simulink model "integrated_controller_scenario5"  (R2021a)
settings: Solver=VariableStepAuto  StartTime=0.0  StopTime=55  RelTol=1e-3
values from neighbouring files (symbols this model uses):
  Cf = 155494.663    [integrated_controller_init.m]    (also in integrated_controller_init_q3.m; integrated_controller_init_q4.m; integrated_controller_init_q5.m; integrated_controller_init_q6_MRM.m)
  Cr = 1554494.663    [integrated_controller_init.m]    (also in integrated_controller_init_q3.m; integrated_controller_init_q4.m; integrated_controller_init_q5.m; integrated_controller_init_q6_MRM.m)
  Iz = 1436.24    [integrated_controller_init.m]    (also in integrated_controller_init_q3.m; integrated_controller_init_q4.m; integrated_controller_init_q5.m; integrated_controller_init_q6_MRM.m)
  L = 3.5    [alc_pathplanning.m]    (also in integrated_controller_init.m = 4.7; integrated_controller_init_q3.m = 4.7; integrated_controller_init_q4.m = 4.7; integrated_controller_init_q5.m = 4.7)
  ld = 10    [integrated_controller_init.m]    (also in integrated_controller_init_q3.m; integrated_controller_init_q4.m; integrated_controller_init_q5.m; integrated_controller_init_q6_MRM.m)
  lf = 1.165    [integrated_controller_init.m]    (also in integrated_controller_init_q3.m; integrated_controller_init_q4.m; integrated_controller_init_q5.m; integrated_controller_init_q6_MRM.m)
  lr = 1.165    [integrated_controller_init.m]    (also in integrated_controller_init_q3.m; integrated_controller_init_q4.m; integrated_controller_init_q5.m; integrated_controller_init_q6_MRM.m)
  m = 1140    [integrated_controller_init.m]    (also in integrated_controller_init_q3.m; integrated_controller_init_q4.m; integrated_controller_init_q5.m; integrated_controller_init_q6_MRM.m)
  md = get_curvature(Vx,yaw_rate_pose,tRef')    [integrated_controller_init.m]    (also in integrated_controller_init_q3.m; integrated_controller_init_q4.m; integrated_controller_init_q5.m; integrated_controller_init_q6_MRM.m)
  Ts = 0.1    [integrated_controller_init.m]    (also in integrated_controller_init_q3.m; integrated_controller_init_q4.m; integrated_controller_init_q5.m; integrated_controller_init_q6_MRM.m)
  V_initial = 15    [integrated_controller_init.m]    (also in integrated_controller_init_q3.m = 11; integrated_controller_init_q4.m = 25; integrated_controller_init_q5.m; integrated_controller_init_q6_MRM.m)
  Vx = a(2) + 2*a(3)*t + 3*a(4)*t.^2 +4*a(5)*t.^3+ a(6)*t.^4    [alc_pathplanning.m]    (also in integrated_controller_init.m = 18; integrated_controller_init_q3.m = 20; integrated_controller_init_q4.m = 25; integrated_controller_init_q5.m = 15)
  xRef = X_ref    [alc_pathplanning.m]    (also in integrated_controller_init.m = path.xRef; integrated_controller_init_q3.m = path.xRef; integrated_controller_init_q4.m = path.xRef; integrated_controller_init_q5.m = refPose(1,:))
  yRef = Y_ref    [alc_pathplanning.m]    (also in integrated_controller_init.m = path.yRef; integrated_controller_init_q3.m = path.yRef; integrated_controller_init_q4.m = path.yRef; integrated_controller_init_q5.m = refPose(2,:))
undefined symbols (not defined in the file or in its folder): sigbuilder_block
libraries: pid_lib x2, mpclib x1, mpcadaslib x1, robotalgslib x1, autolibshared x1
(part 2 of 2)

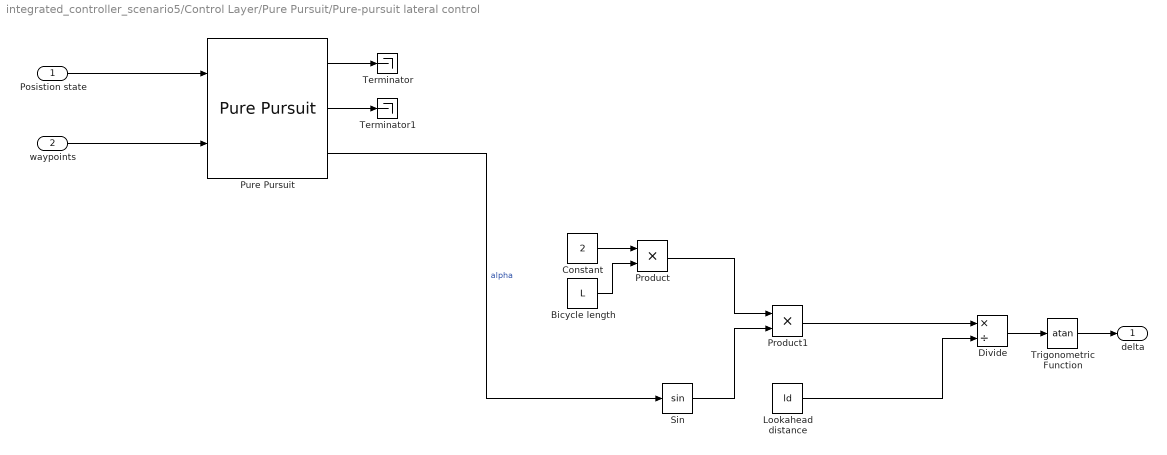
== system integrated_controller_scenario5/Control Layer/Pure Pursuit/Pure-pursuit lateral control ==
  Posistion state : Inport
  waypoints : Inport  Port=2
  Bicycle length : Constant  Value=L
  Constant : Constant  Value=2
  Divide : Product  Inputs=*/
  Lookahead distance : Constant  Value=ld
  Product : Product
  Product1 : Product
  Pure Pursuit : robotalgslib/Pure Pursuit  DesiredLinearVelocity=Vx  MaxAngularVelocity=1.0  LookaheadDistance=ld  TargetDirPort=on  SimulateUsing=Code generation
  Sin : Trigonometry
  Terminator : Terminator
  Terminator1 : Terminator
  Trigonometric Function : Trigonometry  Operator=atan
  delta : Outport
  wires:
  Posistion state/1 -> Pure Pursuit/1
  waypoints/1 -> Pure Pursuit/2
  Pure Pursuit/1 -> Terminator/1
  Pure Pursuit/2 -> Terminator1/1
  Trigonometric Function/1 -> delta/1
  Constant/1 -> Product/1
  Divide/1 -> Trigonometric Function/1
  Lookahead distance/1 -> Divide/2
  Sin/1 -> Product1/2
  Product1/1 -> Divide/1
  Pure Pursuit/3 -> Sin/1  "alpha"
  Bicycle length/1 -> Product/2
  Product/1 -> Product1/1

== system integrated_controller_scenario5/ACC_control_block/ACC_state_logic/Subsystem/If Action Subsystem ==
  v_curve : Inport
  Action Port : ActionPort  ActionPortLabel=if(u1<u2)
  Out1 : Outport
  wires:
  v_curve/1 -> Out1/1

== system integrated_controller_scenario5/ACC_control_block/ACC_state_logic/Subsystem/If Action Subsystem1 ==
  v_limit : Inport
  Action Port : ActionPort  ActionPortLabel=else
  Out1 : Outport
  wires:
  v_limit/1 -> Out1/1

== stateflow chart integrated_controller_scenario5/ACC_control_block/ACC_state_logic/ACC_state_control ==
  state Velocity_and_PSA
    state Velocity_control
      entry: en_man = false;
      en_vel =true;
      en_pos=false;
      en_psa = false;
    state PSA
      entry: en_man = false;
      en_vel =false;
      en_pos=false;
      en_psa = true;
    Velocity_control -> PSA : [v_ideal<v_set]
    (default) -> Velocity_control
    PSA -> Velocity_control : [v_ideal>v_set]
  state Manual_mode
    entry: en_man = true;
    en_vel =false;
    en_pos=false;
  state Headway_control
    entry: en_man = false;
    en_vel =false;
    en_pos=true;
  Manual_mode -> Velocity_and_PSA [order 1] : [(ACC_enable ==1)&&(target_flag==0)]
  Velocity_and_PSA -> Headway_control [order 2] : [(ACC_enable == 1)&(target_flag == 1)&&after(30,sec)]
  Manual_mode -> Headway_control [order 2] : [(ACC_enable == 1) && (target_flag == 1)]
  (default) -> Manual_mode
  Velocity_and_PSA -> Manual_mode [order 1] : [ACC_enable == 0]
  Headway_control -> Velocity_and_PSA [order 2] : [((ACC_enable == 1)&(target_flag==0)|| V_host>commanded_speed + 0.5)&&after(20,sec)]
  Headway_control -> Manual_mode [order 1] : [ACC_enable ==0]
  data: ACC_enable input; V_host input; commanded_speed input; target_flag input; en_man output; en_pos output; en_vel output; en_psa output; v_set input; v_ideal input

== matlab function integrated_controller_scenario5/ACC_control_block/Predictive Speed Assist /MATLAB Function ==
  data: v_limit input; a_max output; v_current input
function a_max = fcn(v_limit,v_current)

if v_current < v_limit+0.2
    a_max = 2000; %mpss
elseif v_current>v_limit+0.2
    a_max = -2000 ; %mpss
else 
    a_max = 0;
    
end

== matlab function integrated_controller_scenario5/Control Layer/MPC/Subsystem/MATLAB Function ==
  settings: updateMethod=DISCRETE  sampleTime=ts
  data: data parameter; seq output; steps parameter; t input; first output; next_t output
function [seq,first,next_t] = fcn(data,steps,t)
%#codegen
[seq,first,next_t] = mpcblock_preview('md',data,steps,t);

== stateflow chart integrated_controller_scenario5/Control Layer/mode manager/Chart ==
  state LCA_off
    entry: en_man = true;
    en_PP = false;
    en_MPC = false;
    en_ALC = false;
  state ALC_on
    entry:en_man = false;
    en_PP = false;
    en_MPC = false;
    en_ALC=true;
  state LCA_On
    state PP
      entry: en_man = false;
      en_PP = true;
      en_MPC = false;
      en_ALC = false;
    state MPC
      entry: en_man = false;
      en_PP = false;
      en_MPC = true;
      en_ALC = false;
    (default) -> PP
    MPC -> PP : [((V_mps <=0.00010) && (Radius >=1000)) ||((V_mps <=0.00010) && (Radius<1000)) ]
    PP -> MPC : [((V_mps >0.00010) && (Radius >=1000)) ||((V_mps >0.00010) && (Radius<1000)) ]
  (default) -> LCA_off
  ALC_on -> LCA_off [order 1] : [(ALC_enable == 0)&&(LCA_enable == 1)]
  LCA_off -> ALC_on [order 2] : [(ALC_enable == 1)&&(LCA_enable == 0)]
  LCA_On -> LCA_off [order 1] : [(LCA_enable ==0)]
  LCA_off -> LCA_On [order 1] : [(LCA_enable ==1)]
  LCA_On -> ALC_on [order 2] : [ALC_enable == 1]
  ALC_on -> LCA_On [order 2] : [ALC_enable == 0]
  data: LCA_enable input; Radius input; V_mps input; en_MPC output; en_PP output; en_man output; en_ALC output; ALC_enable input
